simulink model "rotation_demo_mdl"  (R2025a)
settings: Solver=VariableStepAuto  StartTime=0.0  StopTime=T_end  RelTol=1e-3
values from neighbouring files (symbols this model uses):
  K_AZ = 20    [rotation_demo.m]
  K_PSI = 4 * 2 * mean(abs(R.d_psi)) / (16 * 0.05)    [rotation_demo.m]
  Kd = 4    [rotation_demo.m]
  Kd_psi = 4    [rotation_demo.m]
  Ki = 1.5    [rotation_demo.m]
  Kp = 4    [rotation_demo.m]
  Kp_psi = 4    [rotation_demo.m]
  U_BASE = 0.386    [rotation_demo.m]
  Z_REF = 0.5    [rotation_demo.m]
settings Model: Creator=maximeboulin  LastModifiedBy=maximeboulin

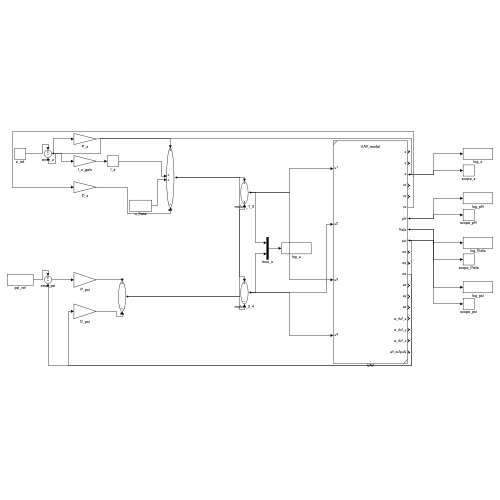
[thumbnail: Simulink's stored preview of the top-level diagram]
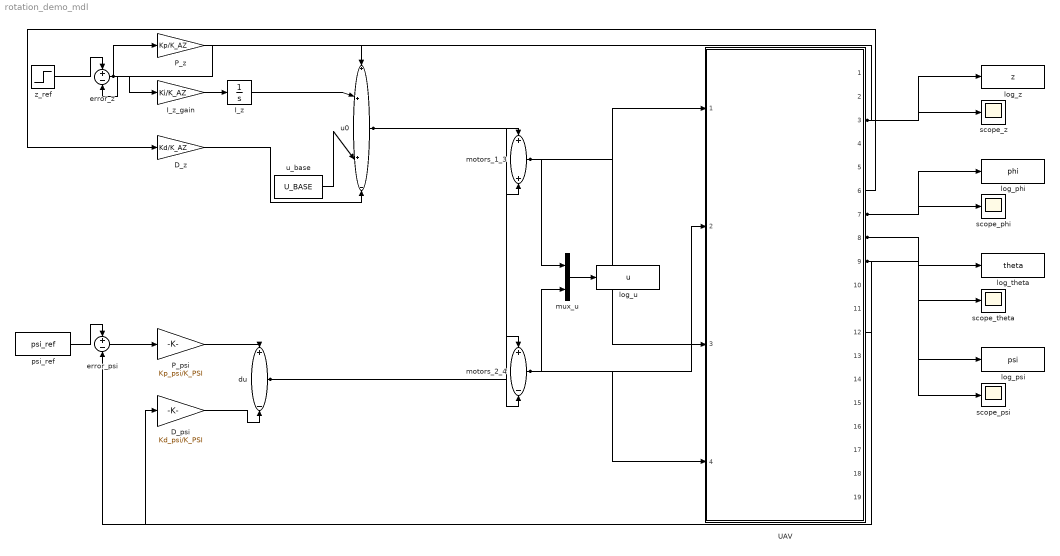
== system rotation_demo_mdl ==
  D_psi : Gain  Gain=Kd_psi/K_PSI
  D_z : Gain  Gain=Kd/K_AZ
  I_z : Integrator
  I_z_gain : Gain  Gain=Ki/K_AZ
  P_psi : Gain  Gain=Kp_psi/K_PSI
  P_z : Gain  Gain=Kp/K_AZ
  UAV : Subsystem  ReferencedSubsystem=UAV_model
  du : Sum  Inputs=+-
  error_psi : Sum  Inputs=+-
  error_z : Sum  Inputs=+-
  log_phi : ToWorkspace  VariableName=phi  SaveFormat=Timeseries  SampleTime=-1
  log_psi : ToWorkspace  VariableName=psi  SaveFormat=Timeseries  SampleTime=-1
  log_theta : ToWorkspace  VariableName=theta  SaveFormat=Timeseries  SampleTime=-1
  log_u : ToWorkspace  VariableName=u  SaveFormat=Timeseries  SampleTime=-1
  log_z : ToWorkspace  VariableName=z  SaveFormat=Timeseries  SampleTime=-1
  motors_1_3 : Sum
  motors_2_4 : Sum  Inputs=+-
  mux_u : Mux  Inputs=2
  psi_ref : FromWorkspace  VariableName=psi_ref
  scope_phi : Scope
  scope_psi : Scope
  scope_theta : Scope
  scope_z : Scope
  u0 : Sum  Inputs=+++-
  u_base : Constant  Value=U_BASE
  z_ref : Step  After=Z_REF  SampleTime=0
  wires:
  z_ref/1 -> error_z/1
  UAV/3 -> error_z/2, log_z/1, scope_z/1
  error_z/1 -> P_z/1, I_z_gain/1
  I_z_gain/1 -> I_z/1
  UAV/6 -> D_z/1
  P_z/1 -> u0/1
  I_z/1 -> u0/2
  u_base/1 -> u0/3
  D_z/1 -> u0/4
  psi_ref/1 -> error_psi/1
  UAV/9 -> error_psi/2, log_psi/1, scope_psi/1
  error_psi/1 -> P_psi/1
  UAV/12 -> D_psi/1
  P_psi/1 -> du/1
  D_psi/1 -> du/2
  u0/1 -> motors_1_3/1, motors_2_4/1
  du/1 -> motors_1_3/2, motors_2_4/2
  motors_1_3/1 -> UAV/1, UAV/3, mux_u/1
  motors_2_4/1 -> UAV/2, UAV/4, mux_u/2
  mux_u/1 -> log_u/1
  UAV/7 -> log_phi/1, scope_phi/1
  UAV/8 -> log_theta/1, scope_theta/1
